simulink model "PX4_Receive"  (R2025b)
settings: Solver=FixedStepAuto  StartTime=0.0  StopTime=60  RelTol=1e-3
undefined symbols (not defined in the file or in its folder): acceleration, actuator, attitude, body_rate, codertarget, command, control, CustomLQR, FlightPlan, from_external, gcbh, HomeNED, HoverThrust, jerk, param1, param2, param3, pitch, pitch_body, position, PX4Params, PX4Tune, q_d, roll, roll_body, source_component, source_system, target_component, target_system, TestAmplitude, TestAxis, thrust_body, timestamp, timestamp_sample, TUNING_ON, TuningMaxClimbRate, TuningMinAltitude, TuningStage, TuningTestStart, velocity, yaw, yaw_body, yaw_sp_move_rate, yawspeed
libraries: px4Utilslib x53, px4uORBlib x52, simulink x13
(part 1 of 2)
settings Model: SimulationMode=external  ExtModeTrigDuration=10  Creator=MarkusKennoHansen  LastModifiedBy=marku
settings SolverCC: PositivePriorityOrder=on  AutoInsertRateTranBlk=on
settings DataIOCC: ReturnWorkspaceOutputs=off
settings OptimizationCC: BlockReduction=off  BooleanDataType=off  EnhancedBackFolding=on  PassReuseOutputArgsAs=Individual arguments  ZeroExternalMemoryAtStartup=off  ZeroInternalMemoryAtStartup=off  MaxStackSize=64  OptimizeBlockOrder=speed  DifferentSizesBufferReuse=on  OptimizationCustomize=off  EfficientTunableParamExpr=on
settings DebuggingCC: SaveWithParameterizedLinksMsg=none  UnderspecifiedInitializationDetection=Classic  MergeDetectMultiDrivingBlocksExec=none  SignalResolutionControl=TryResolveAllWithWarning  IntegerOverflowMsg=none  ParameterPrecisionLossMsg=none  ParameterTunabilityLossMsg=error  IntegerSaturationMsg=none
settings HardwareCC: ProdBitPerPointer=32.0  ProdBitPerSizeT=32.0  ProdBitPerPtrDiffT=32.0  ProdLargestAtomicInteger=Long  ProdLargestAtomicFloat=Double  ProdWordSize=32.0  ProdLongLongMode=on  ProdHWDeviceType=ARM Compatible->ARM Cortex
settings ModelReferenceCC: EnableParallelModelReferenceBuilds=on  PropagateSignalLabelsOutOfModel=off
settings SFSimCC: MATLABDynamicMemAlloc=off  SimTargetLang=C++  SimDLTargetLibrary=mkl-dnn
settings RTWCC: SystemTargetFile=ert.tlc  HardwareBoard=PX4 Host Target  TemplateMakefile=ert_default_tmf  Toolchain=GNU Tools for PX4 Autopilots  PortableWordSizes=on  TargetLang=C++  Description=Embedded Coder
settings CodeAppCC: ForceParamTrailComments=on  IgnoreCustomStorageClasses=off  OperatorAnnotations=on  SimulinkDataObjDesc=on  SFDataObjDesc=on  InsertBlockDesc=on
settings ERTTargetCC: ExtMode=on  ExtModeTransport=2.0  ExtModeStaticAlloc=on  ExtModeMexFile=ext_xcp  ExtModeIntrfLevel=Level2 - Open  InlinedParameterPlacement=Hierarchical

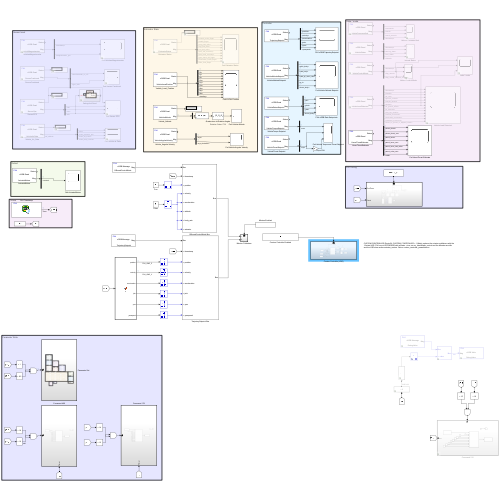
[thumbnail: Simulink's stored preview of the top-level diagram]
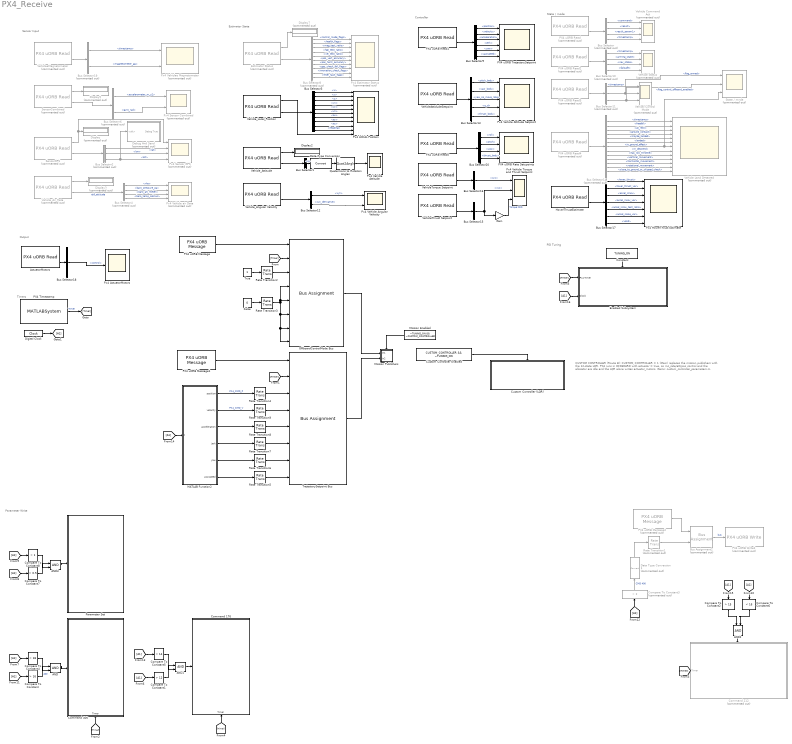
== system PX4_Receive ==
  note: PID Tuning
  note: Timers
  note: Parameter Write
  note: Output
  note: State / mode
  note: Controller
  note: Estimator State
  note: Sensor Input
  note: CUSTOM CONTROLLER (Route B): CUSTOM_CONTROLLER = 1 (Main) replaces the mission publishers with the
      | 12-state LQR. PX4 runs in OFFBOARD with actuator = true, so mc_rate/att/pos_control and the allocator are idle
      | and the LQR alone writes actuator_motors. Gains: custom_controller_parameters.m.
  AND{,1..3} (4 alike) : Logic  IconShape=distinctive  AllPortsSameDT=off  OutDataTypeStr=boolean
  ActuatorMotors : px4uORBlib/PX4 uORB Read  uORBTopic=ActuatorMotors  selectInstance=ActuatorMotors  SampleTime=-1  BlockingMode=off  BlockTimeout=1e-3
  Bus Assignment2 : BusAssignment  Commented=on  AssignedSignals=value
  Bus Selector : BusSelector  Commented=on  OutputSignals=command,result,result_param1,timestamp
  Bus Selector1 : BusSelector  OutputSignals=q
  Bus Selector10 : BusSelector  Commented=on  OutputSignals=timestamp,arming_state,nav_state,failsafe
  Bus Selector11 : BusSelector  Commented=on  OutputSignals=timestamp,flag_armed,flag_control_offboard_enabled
  Bus Selector12 : BusSelector  OutputSignals=xyz,xyz_derivative
  Bus Selector13 : BusSelector  OutputSignals=pitch_body,yaw_body,yaw_sp_move_rate,q_d,thrust_body
  Bus Selector14 : BusSelector  Commented=on  OutputSignals=timestamp,freefall,at_rest,ground_contact,maybe_landed,landed,in_ground_effect,in_descend,has_low_throttle,vertical_movement,horizontal_movement,rotational_movement,close_to_ground_or_skipped_check
  Bus Selector15 : BusSelector  OutputSignals=xyz
  Bus Selector16 : BusSelector  OutputSignals=xyz
  Bus Selector17 : BusSelector  OutputSignals=hover_thrust,hover_thrust_var,accel_innov,accel_innov_var,accel_innov_test_ratio,accel_noise_var,valid
  Bus Selector18 : BusSelector  OutputSignals=control
  Bus Selector19 : BusSelector  Commented=on  OutputSignals=timestamp,magnetometer_ga
  Bus Selector2 : BusSelector  Commented=on  OutputSignals=lat,lon,alt
  Bus Selector20 : BusSelector  OutputSignals=roll,pitch,yaw,thrust_body
  Bus Selector3 : BusSelector  OutputSignals=x,y,z,vx,vy,vz,ax,ay,az,heading
  Bus Selector4 : BusSelector  Commented=on  OutputSignals=rho,baro_pressure_pa,baro_alt_meter,baro_temp_celcius
  Bus Selector6 : BusSelector  Commented=on  OutputSignals=accelerometer_m_s2,gyro_rad
  Bus Selector8 : BusSelector  Commented=on  OutputSignals=control_mode_flags,health_flags,mag_test_ratio,hgt_test_ratio,vel_test_ratio,pos_vert_accuracy,pos_horiz_accuracy,gps_check_fail_flags,innovation_check_flags,filter_fault_flags
  Bus Selector9 : BusSelector  OutputSignals=position,velocity,acceleration,jerk,yaw,yawspeed
  Command 176 : Subsystem
  Command 212 : Subsystem  Commented=on
  Command 400 : Subsystem
  Compare To Constant : simulink/Logic and Bit Operations/Compare To Constant  relop=>  const=16  OutDataTypeStr=boolean
  Compare To Constant1 : simulink/Logic and Bit Operations/Compare To Constant  relop=>  const=12  OutDataTypeStr=boolean
  Compare To Constant2 : simulink/Logic and Bit Operations/Compare To Constant  relop=>  const=15  OutDataTypeStr=boolean
  Compare To Constant3 : simulink/Logic and Bit Operations/Compare To Constant  Commented=on  relop=>  const=2  OutDataTypeStr=boolean
  Compare To Constant4 : simulink/Logic and Bit Operations/Compare To Constant  relop=<  const=18  OutDataTypeStr=boolean
  Compare To Constant5 : simulink/Logic and Bit Operations/Compare To Constant  relop=<  const=14  OutDataTypeStr=boolean
  Compare To Constant6 : simulink/Logic and Bit Operations/Compare To Constant  relop=<  const=16  OutDataTypeStr=boolean
  Compare To Constant7 : simulink/Logic and Bit Operations/Compare To Constant  relop=>  const=0.5  OutDataTypeStr=boolean
  Compare To Constant8 : simulink/Logic and Bit Operations/Compare To Constant  relop=<  const=1  OutDataTypeStr=boolean
  Constant : Constant  Value=TUNING_ON
  Custom Controller (LQR) : Subsystem
  Custom Controller Enabled : Constant  Value=CUSTOM_CONTROLLER && ~TUNING_ON  OutDataTypeStr=boolean
  Data Type Conversion : DataTypeConversion  SaturateOnIntegerOverflow=off  RndMeth=Floor
  Data Type Conversion1 : DataTypeConversion  Commented=on  SaturateOnIntegerOverflow=off  RndMeth=Floor
  Debug And Send : Subsystem  Commented=on
  Digital Clock : DigitalClock  SampleTime=0.01
  Display{,3,5,7} (4 alike) : Display  Commented=on
  Display2 : Display
  Enabled Subsystem : Subsystem  TreatAsAtomicUnit=on
  Estimator Status : px4uORBlib/PX4 uORB Read  Commented=on  uORBTopic=EstimatorStatus  selectInstance=EstimatorStatus  SampleTime=-1  BlockingMode=off  BlockTimeout=1e-3
  False : Constant  Value=0  OutDataTypeStr=Inherit: Inherit via back propagation
  Gain : Gain  Gain=[1 -1 -1]
  HoverThrustEstimate : px4uORBlib/PX4 uORB Read  uORBTopic=HoverThrustEstimate  selectInstance=HoverThrustEstimate  SampleTime=-1  BlockingMode=off  BlockTimeout=1e-3
  MATLAB Function2 : MATLAB Function  TreatAsAtomicUnit=on
  Mission Enabled : Constant  Value=~TUNING_ON && ~CUSTOM_CONTROLLER  OutDataTypeStr=boolean
  Mission Publishers : Subsystem
  OffboardControlMode Bus : BusAssignment  AssignedSignals=timestamp,position,velocity,acceleration,attitude,body_rate,actuator
  PX4 Timestamp : MATLABSystem  InitFcn=codertarget.pixhawk.internal.registration.registerBlockInResourceMgr(gcbh,'PX4_Timestamp');  System=px4.internal.block.getPX4AbsoluteTime  SampleTime=0.01
  PX4 uORB Message : px4uORBlib/PX4 uORB Message  uORBTopic=OffboardControlMode  SampleTime=-1  selectInstance=OffboardControlMode
  PX4 uORB Message1 : px4uORBlib/PX4 uORB Message  uORBTopic=TrajectorySetpoint  SampleTime=-1  selectInstance=TrajectorySetpoint
  PX4 uORB Message2 : px4uORBlib/PX4 uORB Message  Commented=on  uORBTopic=DebugValue  SampleTime=-1  selectInstance=DebugValue
  PX4 uORB Rate Setupoints : Scope  NumInputPorts=4
      settings: ActiveDisplayYMinimum=-4.7996553778648376  ActiveDisplayYMaximum=4.7996553778648376  DataLoggingVariableName=ScopeData22
  PX4 uORB Read : px4uORBlib/PX4 uORB Read  Commented=on  uORBTopic=VehicleCommandAck  selectInstance=VehicleCommandAck  SampleTime=-1  BlockingMode=off  BlockTimeout=1e-3
  PX4 uORB Read1 : px4uORBlib/PX4 uORB Read  uORBTopic=TrajectorySetpoint  selectInstance=TrajectorySetpoint  SampleTime=-1  BlockingMode=off  BlockTimeout=1e-3
  PX4 uORB Read2 : px4uORBlib/PX4 uORB Read  Commented=on  uORBTopic=VehicleStatus  selectInstance=VehicleStatus  SampleTime=-1  BlockingMode=off  BlockTimeout=1e-3
  PX4 uORB Read3 : px4uORBlib/PX4 uORB Read  Commented=on  uORBTopic=VehicleControlMode  selectInstance=VehicleControlMode  SampleTime=-1  BlockingMode=off  BlockTimeout=1e-3
  PX4 uORB Read4 : px4uORBlib/PX4 uORB Read  Commented=on  uORBTopic=VehicleLandDetected  selectInstance=VehicleLandDetected  SampleTime=-1  BlockingMode=off  BlockTimeout=1e-3
  PX4 uORB Read5 : px4uORBlib/PX4 uORB Read  uORBTopic=VehicleRatesSetpoint  selectInstance=VehicleRatesSetpoint  SampleTime=-1  BlockingMode=off  BlockTimeout=1e-3
  PX4 uORB TrajectorySetpoint : Scope  NumInputPorts=6
      settings: ActiveDisplayYMinimum=-0.034024091670289636  ActiveDisplayYMaximum=0.16679841303266585  DataLoggingVariableName=ScopeData13
  PX4 uORB Write2 : px4uORBlib/PX4 uORB Write  Commented=on  uORBTopic=DebugValue  selectInstance=DebugValue  MessageQueueLen=1
  Parameter Set : Subsystem
  Px4 ActuatorMotors : Scope
      settings: ActiveDisplayYMinimum=-0.12499999999999997  ActiveDisplayYMaximum=1.125  DataLoggingVariableName=ScopeData20
  "Px4 Estimator Status " : Scope  Commented=on  NumInputPorts=10
      settings: ActiveDisplayString=3  ActiveDisplayYMinimum=-0.00022157638159114862  ActiveDisplayYMaximum=0.0019941874343203381  DataLoggingVariableName=ScopeData7
  Px4 HoverThrust Estimate : Scope  NumInputPorts=7
      settings: ActiveDisplayYMinimum=-1  ActiveDisplayYMaximum=1  DataLoggingVariableName=ScopeData19
  Px4 LOCAL Position : Scope  NumInputPorts=11
      settings: ActiveDisplayYMinimum=-0.0066038075601682067  ActiveDisplayYMaximum=0.015251552104018629  DataLoggingVariableName=ScopeData3
  Px4 Sensor Combined : Scope  Commented=on  NumInputPorts=2
      settings: ActiveDisplayYMinimum=-34.435865640640259  ActiveDisplayYMaximum=33.0942919254303  DataLoggingVariableName=ScopeData6
  Px4 Sensor GPS : Scope  Commented=on  NumInputPorts=4
      settings: ActiveDisplayString=3  ActiveDisplayYMinimum=1.25208830125E+8  ActiveDisplayYMaximum=1.25210948875E+8
  Px4 Vehiclae Magnetometer : Scope  Commented=on  NumInputPorts=2
      settings: ActiveDisplayYMinimum=-0.399243738502264  ActiveDisplayYMaximum=0.3986239992082119  DataLoggingVariableName=ScopeData21
  Px4 Vehicle Angular Velocity : Scope  NumInputPorts=2
      settings: ActiveDisplayYMinimum=-617.98886871337891  ActiveDisplayYMaximum=742.34903717041016  DataLoggingVariableName=ScopeData15
  Px4 Vehicle Attitude : Scope
      settings: ActiveDisplayYMinimum=-3.9110912623215079  ActiveDisplayYMaximum=3.91992136617894  DataLoggingVariableName=ScopeData2
  Px4 Vehicle Attitude Setpoint : Scope  NumInputPorts=5
      settings: ActiveDisplayYMinimum=1.739683210849762  ActiveDisplayYMaximum=1.742851197719574  DataLoggingVariableName=ScopeData16
  Px4 Vehicle Torque and Thrust Setpoint : Scope  NumInputPorts=3
      settings: ActiveDisplayYMinimum=-0.20918363705277443  ActiveDisplayYMaximum=0.023242626339197155  DataLoggingVariableName=ScopeData18
  Px4 Vehicle air Data : Scope  Commented=on  NumInputPorts=4
      settings: ActiveDisplayString=3  ActiveDisplayYMinimum=0.95836924761533737  ActiveDisplayYMaximum=0.99945063143968582  DataLoggingVariableName=ScopeData4
  Quaternions to Rotation Angles : Quat2Angle
      settings: AttributesFormatString=Rotation Order: %<rotationOrder>
  Rate Transition1 : RateTransition  Commented=on  OutPortSampleTime=1/500
  Rate Transition{2..9} (8 alike) : RateTransition  Deterministic=off  OutPortSampleTime=0.01
  SensorCombined : px4uORBlib/PX4 uORB Read  Commented=on  uORBTopic=SensorCombined  selectInstance=SensorCombined  SampleTime=-1  BlockingMode=off  BlockTimeout=1e-3
  SensorGPS : px4uORBlib/PX4 uORB Read  Commented=on  uORBTopic=SensorGps  selectInstance=sensor_gps  SampleTime=-1  BlockingMode=off  BlockTimeout=1e-3
  State / mode : Scope  Commented=on  NumInputPorts=3
      settings: DataLoggingVariableName=ScopeData23
  TrajectorySetpoint Bus : BusAssignment  AssignedSignals=timestamp,position,velocity,acceleration,jerk,yaw,yawspeed
  True : Constant  OutDataTypeStr=Inherit: Inherit via back propagation
  Vehical Control Mode : Scope  Commented=on  NumInputPorts=3
      settings: ActiveDisplayYMinimum=3.7235000000000009E+6  ActiveDisplayYMaximum=4.56485E+7  DataLoggingVariableName=ScopeData14
  Vehical Status : Scope  Commented=on  NumInputPorts=4
      settings: ActiveDisplayYMinimum=833500.00000000093  ActiveDisplayYMaximum=3.56185E+7  DataLoggingVariableName=ScopeData8
  VehiclaeMagnetometer : px4uORBlib/PX4 uORB Read  Commented=on  uORBTopic=VehicleMagnetometer  selectInstance=VehicleMagnetometer  SampleTime=-1  BlockingMode=off  BlockTimeout=1e-3
  Vehicle Command Ack : Scope  Commented=on  NumInputPorts=4
      settings: ActiveDisplayYMinimum=-49.999999999999986  ActiveDisplayYMaximum=450  DataLoggingVariableName=ScopeData12
  Vehicle Land Detected : Scope  Commented=on  NumInputPorts=13
      settings: ActiveDisplayYMinimum=3.0415000000000009E+6  ActiveDisplayYMaximum=4.55065E+7  DataLoggingVariableName=ScopeData17
  VehicleAttidudeSetpoint : px4uORBlib/PX4 uORB Read  uORBTopic=VehicleAttitudeSetpoint  selectInstance=vehicle_attitude_setpoint  SampleTime=-1  BlockingMode=off  BlockTimeout=1e-3
  VehicleThrust Setpoint : px4uORBlib/PX4 uORB Read  uORBTopic=VehicleThrustSetpoint  selectInstance=vehicle_thrust_setpoint  SampleTime=-1  BlockingMode=off  BlockTimeout=1e-3
  VehicleTorque Setpoint : px4uORBlib/PX4 uORB Read  uORBTopic=VehicleTorqueSetpoint  selectInstance=vehicle_torque_setpoint  SampleTime=-1  BlockingMode=off  BlockTimeout=1e-3
  Vehicle_Air_Data : px4uORBlib/PX4 uORB Read  Commented=on  uORBTopic=VehicleAirData  selectInstance=VehicleAirData  SampleTime=-1  BlockingMode=off  BlockTimeout=1e-3
  Vehicle_Angular Velocity : px4uORBlib/PX4 uORB Read  uORBTopic=VehicleAngularVelocity  selectInstance=vehicle_angular_velocity  SampleTime=-1  BlockingMode=off  BlockTimeout=1e-3
  Vehicle_Attitude : px4uORBlib/PX4 uORB Read  uORBTopic=VehicleAttitude  selectInstance=vehicle_attitude  SampleTime=-1  BlockingMode=off  BlockTimeout=1e-3
  Vehicle_Local_Position : px4uORBlib/PX4 uORB Read  uORBTopic=VehicleLocalPosition  selectInstance=vehicle_local_position  SampleTime=-1  BlockingMode=off  BlockTimeout=1e-3
  wires:
  Bus Selector2/2 -> Px4 Sensor GPS/3  "<lon>"
  Bus Selector2/3 -> Px4 Sensor GPS/4, Debug And Send/1(<alt>)  "<alt>"
  Bus Selector2/1 -> Px4 Sensor GPS/2  "<lat>"
  SensorGPS/1 -> Display/1, Px4 Sensor GPS/1
  SensorGPS/2 -> Bus Selector2/1
  Vehicle_Attitude/2 -> Bus Selector1/1
  Vehicle_Local_Position/2 -> Bus Selector3/1
  Bus Selector1/1 -> Data Type Conversion/1  "<q>"
  Quaternions to Rotation Angles/1 -> Px4 Vehicle Attitude/1
  Data Type Conversion/1 -> Quaternions to Rotation Angles/1
  Vehicle_Attitude/1 -> Display2/1
  Rate Transition2/1 -> OffboardControlMode Bus/3
  Rate Transition9/1 -> TrajectorySetpoint Bus/4
  Rate Transition7/1 -> TrajectorySetpoint Bus/6
  Rate Transition4/1 -> TrajectorySetpoint Bus/3
  PX4 uORB Message1/1 -> TrajectorySetpoint Bus/1
  False/1 -> Rate Transition3/1
  PX4 uORB Message/1 -> OffboardControlMode Bus/1
  MATLAB Function2/4(jerk) -> Rate Transition7/1
  True/1 -> Rate Transition2/1
  Rate Transition5/1 -> TrajectorySetpoint Bus/8
  Rate Transition3/1 -> OffboardControlMode Bus/7, OffboardControlMode Bus/8, OffboardControlMode Bus/6, OffboardControlMode Bus/4, OffboardControlMode Bus/5
  Rate Transition6/1 -> TrajectorySetpoint Bus/7
  Rate Transition8/1 -> TrajectorySetpoint Bus/5
  PX4 uORB Read/2 -> Bus Selector/1
  Bus Selector/1 -> Vehicle Command Ack/1  "<command>"
  Bus Selector/2 -> Vehicle Command Ack/2  "<result>"
  Bus Selector/3 -> Vehicle Command Ack/3  "<result_param1>"
  Bus Selector/4 -> Vehicle Command Ack/4  "<timestamp>"
  Bus Assignment2/1 -> PX4 uORB Write2/1  "bus"
  PX4 uORB Message2/1 -> Bus Assignment2/1
  Rate Transition1/1 -> Bus Assignment2/2
  Data Type Conversion1/1 -> Rate Transition1/1
  PX4 uORB Read1/2 -> Bus Selector9/1
  Bus Selector9/1 -> PX4 uORB TrajectorySetpoint/1  "<position>"
  Bus Selector9/2 -> PX4 uORB TrajectorySetpoint/2  "<velocity>"
  Bus Selector9/3 -> PX4 uORB TrajectorySetpoint/3  "<acceleration>"
  Bus Selector9/4 -> PX4 uORB TrajectorySetpoint/4  "<jerk>"
  Bus Selector9/5 -> PX4 uORB TrajectorySetpoint/5  "<yaw>"
  Bus Selector9/6 -> PX4 uORB TrajectorySetpoint/6  "<yawspeed>"
  Compare To Constant3/1 -> Data Type Conversion1/1  "CMD 400"
  AND/1 -> Command 400/Trigger
  Compare To Constant/1 -> AND/1  "400"
  Compare To Constant4/1 -> AND/2
  AND1/1 -> Command 176/Trigger
  Compare To Constant1/1 -> AND1/1
  Compare To Constant5/1 -> AND1/2
  Compare To Constant2/1 -> AND2/1
  AND2/1 -> Command 212/Trigger
  Compare To Constant6/1 -> AND2/2
  Compare To Constant7/1 -> AND3/1
  Compare To Constant8/1 -> AND3/2
  AND3/1 -> Parameter Set/Trigger
  PX4 uORB Read2/2 -> Bus Selector10/1
  Bus Selector10/1 -> Vehical Status/1  "<timestamp>"
  Bus Selector10/3 -> Vehical Status/3  "<nav_state>"
  Bus Selector10/4 -> Vehical Status/4  "<failsafe>"
  PX4 uORB Read3/2 -> Bus Selector11/1
  Bus Selector10/2 -> Vehical Status/2  "<arming_state>"
  Bus Selector11/1 -> Vehical Control Mode/1  "<timestamp>"
  Bus Selector11/2 -> State / mode/1, Vehical Control Mode/2  "<flag_armed>"
  Bus Selector11/3 -> State / mode/2, Vehical Control Mode/3  "<flag_control_offboard_enabled>"
  Vehicle_Angular Velocity/2 -> Bus Selector12/1
  Bus Selector12/1 -> Px4 Vehicle Angular Velocity/1  "<xyz>"
  Bus Selector12/2 -> Px4 Vehicle Angular Velocity/2  "<xyz_derivative>"
  VehicleAttidudeSetpoint/2 -> Bus Selector13/1
  Bus Selector13/1 -> Px4 Vehicle Attitude Setpoint/1  "<pitch_body>"
  Bus Selector13/2 -> Px4 Vehicle Attitude Setpoint/2  "<yaw_body>"
  Bus Selector13/3 -> Px4 Vehicle Attitude Setpoint/3  "<yaw_sp_move_rate>"
  Bus Selector13/4 -> Px4 Vehicle Attitude Setpoint/4  "<q_d>"
  Bus Selector13/5 -> Px4 Vehicle Attitude Setpoint/5  "<thrust_body>"
  PX4 uORB Read4/2 -> Bus Selector14/1
  Bus Selector14/1 -> Vehicle Land Detected/1  "<timestamp>"
  Bus Selector14/2 -> Vehicle Land Detected/2  "<freefall>"
  Bus Selector14/3 -> Vehicle Land Detected/3  "<at_rest>"
  Bus Selector14/4 -> Vehicle Land Detected/4  "<ground_contact>"
  Bus Selector14/5 -> Vehicle Land Detected/5  "<maybe_landed>"
  Bus Selector14/6 -> Vehicle Land Detected/6  "<landed>"
  Bus Selector14/7 -> State / mode/3, Vehicle Land Detected/7  "<in_ground_effect>"
  Bus Selector14/8 -> Vehicle Land Detected/8  "<in_descend>"
  Bus Selector14/9 -> Vehicle Land Detected/9  "<has_low_throttle>"
  Bus Selector14/10 -> Vehicle Land Detected/10  "<vertical_movement>"
  Bus Selector14/11 -> Vehicle Land Detected/11  "<horizontal_movement>"
  Bus Selector14/12 -> Vehicle Land Detected/12  "<rotational_movement>"
  Bus Selector14/13 -> Vehicle Land Detected/13  "<close_to_ground_or_skipped_check>"
  VehicleThrust Setpoint/2 -> Bus Selector15/1
  VehicleTorque Setpoint/2 -> Bus Selector16/1
  HoverThrustEstimate/2 -> Bus Selector17/1
  Bus Selector16/1 -> Px4 Vehicle Torque and Thrust Setpoint/1  "<xyz>"
  Bus Selector15/1 -> Gain/1, Px4 Vehicle Torque and Thrust Setpoint/2  "<xyz>"
  Bus Selector17/1 -> Px4 HoverThrust Estimate/1  "<hover_thrust>"
  Bus Selector17/2 -> Px4 HoverThrust Estimate/2  "<hover_thrust_var>"
  Bus Selector17/3 -> Px4 HoverThrust Estimate/3  "<accel_innov>"
  Bus Selector17/4 -> Px4 HoverThrust Estimate/4  "<accel_innov_var>"
  Bus Selector17/5 -> Px4 HoverThrust Estimate/5  "<accel_innov_test_ratio>"
  Bus Selector17/6 -> Px4 HoverThrust Estimate/6  "<accel_noise_var>"
  Bus Selector17/7 -> Px4 HoverThrust Estimate/7  "<valid>"
  Bus Selector6/1 -> Px4 Sensor Combined/1  "<accelerometer_m_s2>"
  Bus Selector6/2 -> Px4 Sensor Combined/2  "<gyro_rad>"
  SensorCombined/1 -> Display5/1
  SensorCombined/2 -> Bus Selector6/1
  ActuatorMotors/2 -> Bus Selector18/1
  VehiclaeMagnetometer/2 -> Bus Selector19/1
  Bus Selector19/1 -> Px4 Vehiclae Magnetometer/1  "<timestamp>"
  Bus Selector19/2 -> Px4 Vehiclae Magnetometer/2  "<magnetometer_ga>"
  Bus Selector4/2 -> Px4 Vehicle air Data/2  "<baro_pressure_pa>"
  Vehicle_Air_Data/2 -> Bus Selector4/1  "ekf_attitude"
  Bus Selector4/3 -> Px4 Vehicle air Data/3  "<baro_alt_meter>"
  Vehicle_Air_Data/1 -> Display3/1
  Bus Selector4/4 -> Px4 Vehicle air Data/4  "<baro_temp_celcius>"
  Bus Selector4/1 -> Px4 Vehicle air Data/1  "<rho>"
  Bus Selector8/10 -> "Px4 Estimator Status "/10  "<filter_fault_flags>"
  Bus Selector8/8 -> "Px4 Estimator Status "/8  "<gps_check_fail_flags>"
  Bus Selector8/9 -> "Px4 Estimator Status "/9  "<innovation_check_flags>"
  Estimator Status/2 -> Bus Selector8/1
  Estimator Status/1 -> Display7/1
  Bus Selector8/1 -> "Px4 Estimator Status "/1  "<control_mode_flags>"
  Bus Selector8/5 -> "Px4 Estimator Status "/5  "<vel_test_ratio>"
  Bus Selector8/3 -> "Px4 Estimator Status "/3  "<mag_test_ratio>"
  Bus Selector8/7 -> "Px4 Estimator Status "/7  "<pos_horiz_accuracy>"
  Bus Selector8/6 -> "Px4 Estimator Status "/6  "<pos_vert_accuracy>"
  Bus Selector8/4 -> "Px4 Estimator Status "/4  "<hgt_test_ratio>"
  Bus Selector8/2 -> "Px4 Estimator Status "/2  "<health_flags>"
  PX4 uORB Read5/2 -> Bus Selector20/1
  Bus Selector20/1 -> PX4 uORB Rate Setupoints/1  "<roll>"
  Bus Selector20/2 -> PX4 uORB Rate Setupoints/2  "<pitch>"
  Bus Selector20/3 -> PX4 uORB Rate Setupoints/3  "<yaw>"
  Bus Selector20/4 -> PX4 uORB Rate Setupoints/4  "<thrust_body>"
  Bus Selector18/1 -> Px4 ActuatorMotors/1  "<control>"
  Gain/1 -> Px4 Vehicle Torque and Thrust Setpoint/3  "Torque FRD"
  MATLAB Function2/1(position) -> Rate Transition4/1  "PX4_CMD_P"
  Bus Selector3/1 -> Px4 LOCAL Position/1  "<x>"
  Bus Selector3/2 -> Px4 LOCAL Position/2  "<y>"
  Bus Selector3/3 -> Px4 LOCAL Position/3  "<z>"
  Bus Selector3/4 -> Px4 LOCAL Position/4  "<vx>"
  Bus Selector3/5 -> Px4 LOCAL Position/5  "<vy>"
  Bus Selector3/6 -> Px4 LOCAL Position/6  "<vz>"
  Bus Selector3/7 -> Px4 LOCAL Position/7  "<ax>"
  Bus Selector3/8 -> Px4 LOCAL Position/8  "<ay>"
  Bus Selector3/9 -> Px4 LOCAL Position/9  "<az>"
  Bus Selector3/10 -> Px4 LOCAL Position/10  "<heading>"
  Vehicle_Local_Position/1 -> Px4 LOCAL Position/11
  MATLAB Function2/2(velocity) -> Rate Transition9/1  "PX4_CMD_V"
  MATLAB Function2/3(acceleration) -> Rate Transition8/1
  MATLAB Function2/5(yaw) -> Rate Transition6/1
  MATLAB Function2/6(yawspeed) -> Rate Transition5/1
  Constant/1 -> Enabled Subsystem/Enable
  PX4 Timestamp/1 -> [Timer]  "Timer"
  [Timer] -> OffboardControlMode Bus/2
  [Timer] -> TrajectorySetpoint Bus/2
  [Timer] -> Command 400/1(Timer)
  [Timer] -> Command 212/1(Timer)
  [Timer] -> Command 176/1(Timer)
  [Timer] -> Enabled Subsystem/1(Px4 Timer)
  Digital Clock/1 -> [A1]
  [A1] -> Compare To Constant1/1
  [A1] -> Compare To Constant4/1
  [A1] -> Compare To Constant7/1
  [A1] -> Compare To Constant8/1
  [A1] -> Compare To Constant6/1
  [A1] -> Compare To Constant/1
  [A1] -> Compare To Constant3/1
  [A1] -> Compare To Constant5/1
  [A1] -> MATLAB Function2/1(t)
  [A1] -> Compare To Constant2/1
  [A1] -> Enabled Subsystem/2(Clock)
  OffboardControlMode Bus/1 -> Mission Publishers/1(In1)
  TrajectorySetpoint Bus/1 -> Mission Publishers/2(In2)
  Mission Enabled/1 -> Mission Publishers/Enable
  Custom Controller Enabled/1 -> Custom Controller (LQR)/Enable

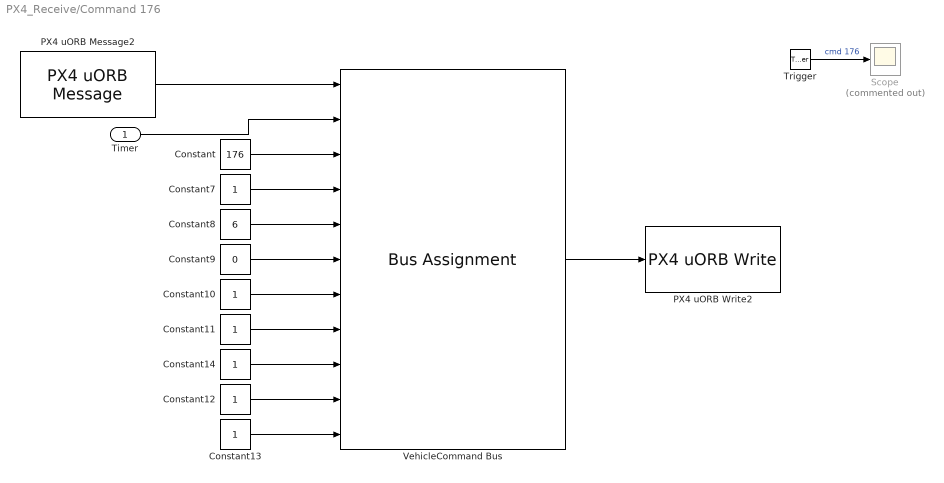
== system PX4_Receive/Command 176 ==
  Timer : Inport
  Trigger : TriggerPort  VariantControl=(inherit)  ShowOutputPort=on  PortDimensions=1
  Constant : Constant  Value=176  OutDataTypeStr=Inherit: Inherit via back propagation  SampleTime=-1
  Constant{7,10..14} (6 alike) : Constant  OutDataTypeStr=Inherit: Inherit via back propagation  SampleTime=-1
  Constant8 : Constant  Value=6  OutDataTypeStr=Inherit: Inherit via back propagation  SampleTime=-1
  Constant9 : Constant  Value=0  OutDataTypeStr=Inherit: Inherit via back propagation  SampleTime=-1
  PX4 uORB Message2 : px4uORBlib/PX4 uORB Message  uORBTopic=VehicleCommand  SampleTime=-1  selectInstance=vehicle_command
  PX4 uORB Write2 : px4uORBlib/PX4 uORB Write  uORBTopic=VehicleCommand  selectInstance=vehicle_command  MessageQueueLen=1
  Scope : Scope  Commented=on
      settings: ActiveDisplayYMinimum=-0.12499999999999997  ActiveDisplayYMaximum=1.125  DataLoggingVariableName=ScopeData10
  VehicleCommand Bus : BusAssignment  AssignedSignals=timestamp,command,param1,param2,param3,target_system,target_component,source_system,source_component,from_external
  wires:
  Constant7/1 -> VehicleCommand Bus/4
  Constant12/1 -> VehicleCommand Bus/10
  Constant11/1 -> VehicleCommand Bus/8
  Constant10/1 -> VehicleCommand Bus/7
  VehicleCommand Bus/1 -> PX4 uORB Write2/1
  Constant14/1 -> VehicleCommand Bus/9
  Constant13/1 -> VehicleCommand Bus/11
  Constant8/1 -> VehicleCommand Bus/5
  PX4 uORB Message2/1 -> VehicleCommand Bus/1
  Constant9/1 -> VehicleCommand Bus/6
  Constant/1 -> VehicleCommand Bus/3
  Trigger/1 -> Scope/1  "cmd 176"
  Timer/1 -> VehicleCommand Bus/2

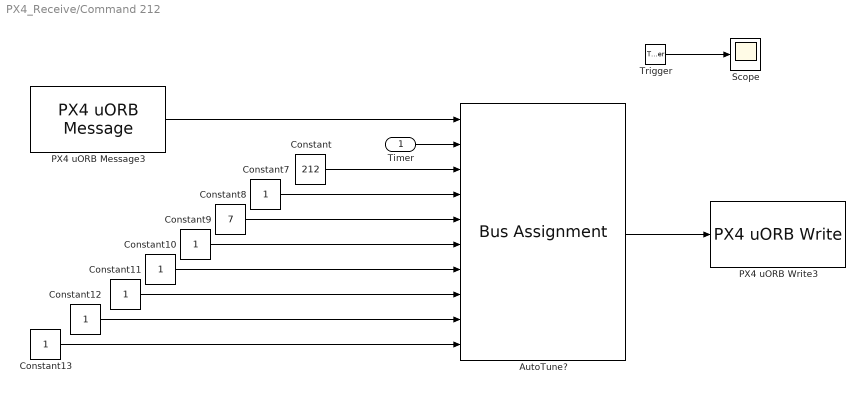
== system PX4_Receive/Command 212 ==
  Timer : Inport
  Trigger : TriggerPort  VariantControl=(inherit)  ShowOutputPort=on  PortDimensions=1
  AutoTune? : BusAssignment  AssignedSignals=timestamp,command,param1,param2,target_system,target_component,source_system,source_component,from_external
  Constant : Constant  Value=212  OutDataTypeStr=Inherit: Inherit via back propagation
  Constant{7,9..13} (6 alike) : Constant  OutDataTypeStr=Inherit: Inherit via back propagation
  Constant8 : Constant  Value=7  OutDataTypeStr=Inherit: Inherit via back propagation
  PX4 uORB Message3 : px4uORBlib/PX4 uORB Message  uORBTopic=VehicleCommand  SampleTime=-1  selectInstance=vehicle_command
  PX4 uORB Write3 : px4uORBlib/PX4 uORB Write  uORBTopic=VehicleCommand  selectInstance=vehicle_command  MessageQueueLen=1
  Scope : Scope
      settings: ActiveDisplayYMinimum=-0.12499999999999997  ActiveDisplayYMaximum=1.125  DataLoggingVariableName=ScopeData11
  wires:
  Trigger/1 -> Scope/1
  Constant12/1 -> AutoTune?/9
  Constant7/1 -> AutoTune?/4
  Constant10/1 -> AutoTune?/7
  Constant8/1 -> AutoTune?/5
  PX4 uORB Message3/1 -> AutoTune?/1
  Constant/1 -> AutoTune?/3
  Constant11/1 -> AutoTune?/8
  Constant9/1 -> AutoTune?/6
  AutoTune?/1 -> PX4 uORB Write3/1
  Constant13/1 -> AutoTune?/10
  Timer/1 -> AutoTune?/2

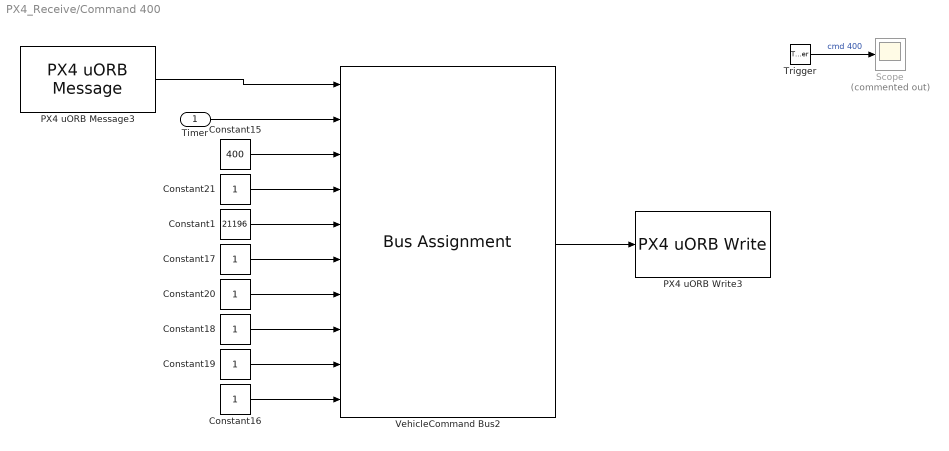
== system PX4_Receive/Command 400 ==
  Timer : Inport
  Trigger : TriggerPort  VariantControl=(inherit)  ShowOutputPort=on  PortDimensions=1
  Constant1 : Constant  Value=21196  OutDataTypeStr=Inherit: Inherit via back propagation  SampleTime=-1
  Constant15 : Constant  Value=400  OutDataTypeStr=Inherit: Inherit via back propagation  SampleTime=-1
  Constant{16..21} (6 alike) : Constant  OutDataTypeStr=Inherit: Inherit via back propagation  SampleTime=-1
  PX4 uORB Message3 : px4uORBlib/PX4 uORB Message  uORBTopic=VehicleCommand  SampleTime=-1  selectInstance=vehicle_command
  PX4 uORB Write3 : px4uORBlib/PX4 uORB Write  uORBTopic=VehicleCommand  selectInstance=vehicle_command  MessageQueueLen=1
  Scope : Scope  Commented=on
      settings: ActiveDisplayYMinimum=-0.12499999999999997  ActiveDisplayYMaximum=1.125  DataLoggingVariableName=ScopeData11
  VehicleCommand Bus2 : BusAssignment  AssignedSignals=timestamp,command,param1,param2,target_system,target_component,source_system,source_component,from_external
  wires:
  Constant21/1 -> VehicleCommand Bus2/4
  PX4 uORB Message3/1 -> VehicleCommand Bus2/1
  VehicleCommand Bus2/1 -> PX4 uORB Write3/1
  Constant17/1 -> VehicleCommand Bus2/6
  Constant20/1 -> VehicleCommand Bus2/7
  Constant19/1 -> VehicleCommand Bus2/9
  Constant18/1 -> VehicleCommand Bus2/8
  Constant15/1 -> VehicleCommand Bus2/3
  Constant16/1 -> VehicleCommand Bus2/10
  Trigger/1 -> Scope/1  "cmd 400"
  Timer/1 -> VehicleCommand Bus2/2
  Constant1/1 -> VehicleCommand Bus2/5

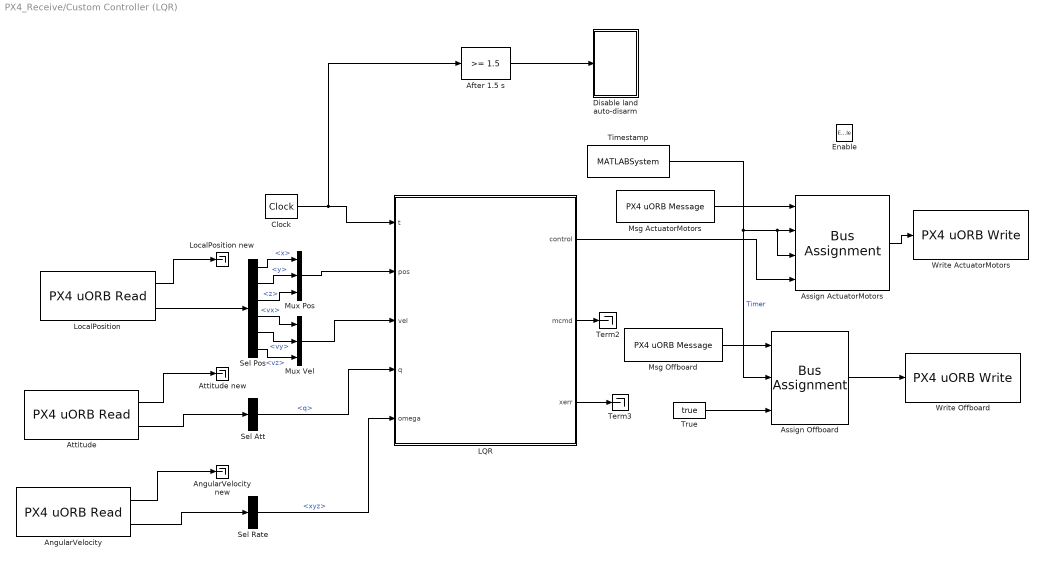
== system PX4_Receive/Custom Controller (LQR) ==
  Enable : EnablePort  StatesWhenEnabling=reset
  After 1.5 s : simulink/Logic and Bit Operations/Compare To Constant  relop=>=  const=1.5  OutDataTypeStr=boolean
  AngularVelocity : px4uORBlib/PX4 uORB Read  uORBTopic=VehicleAngularVelocity  selectInstance=vehicle_angular_velocity  SampleTime=-1  BlockingMode=off  BlockTimeout=1e-3
  AngularVelocity new : Terminator
  Assign ActuatorMotors : BusAssignment  AssignedSignals=timestamp,timestamp_sample,control
  Assign Offboard : BusAssignment  AssignedSignals=timestamp,actuator
  Attitude : px4uORBlib/PX4 uORB Read  uORBTopic=VehicleAttitude  selectInstance=vehicle_attitude  SampleTime=-1  BlockingMode=off  BlockTimeout=1e-3
  Attitude new : Terminator
  Clock : DigitalClock  SampleTime=0.01
  Disable land auto-disarm : Subsystem
  LQR : MATLAB Function  TreatAsAtomicUnit=on
  LocalPosition : px4uORBlib/PX4 uORB Read  uORBTopic=VehicleLocalPosition  selectInstance=vehicle_local_position  SampleTime=-1  BlockingMode=off  BlockTimeout=1e-3
  LocalPosition new : Terminator
  Msg ActuatorMotors : px4uORBlib/PX4 uORB Message  uORBTopic=ActuatorMotors  SampleTime=-1  selectInstance=ActuatorMotors
  Msg Offboard : px4uORBlib/PX4 uORB Message  uORBTopic=OffboardControlMode  SampleTime=-1  selectInstance=OffboardControlMode
  Mux Pos : Mux  Inputs=3
  Mux Vel : Mux  Inputs=3
  Sel Att : BusSelector  OutputSignals=q
  Sel Pos : BusSelector  OutputSignals=x,y,z,vx,vy,vz
  Sel Rate : BusSelector  OutputSignals=xyz
  Term2 : Terminator
  Term3 : Terminator
  Timestamp : MATLABSystem  InitFcn=codertarget.pixhawk.internal.registration.registerBlockInResourceMgr(gcbh,'PX4_Timestamp');  System=px4.internal.block.getPX4AbsoluteTime  SampleTime=0.01
  True : Constant  Value=true  OutDataTypeStr=boolean
  Write ActuatorMotors : px4uORBlib/PX4 uORB Write  uORBTopic=ActuatorMotors  selectInstance=ActuatorMotors  MessageQueueLen=1
  Write Offboard : px4uORBlib/PX4 uORB Write  uORBTopic=OffboardControlMode  selectInstance=OffboardControlMode  MessageQueueLen=1
  wires:
  LocalPosition/1 -> LocalPosition new/1
  Attitude/1 -> Attitude new/1
  AngularVelocity/1 -> AngularVelocity new/1
  LocalPosition/2 -> Sel Pos/1
  Sel Pos/1 -> Mux Pos/1  "<x>"
  Sel Pos/4 -> Mux Vel/1  "<vx>"
  Sel Pos/2 -> Mux Pos/2  "<y>"
  Sel Pos/5 -> Mux Vel/2  "<vy>"
  Sel Pos/3 -> Mux Pos/3  "<z>"
  Sel Pos/6 -> Mux Vel/3  "<vz>"
  Attitude/2 -> Sel Att/1
  AngularVelocity/2 -> Sel Rate/1
  Clock/1 -> LQR/1(t), After 1.5 s/1
  Mux Pos/1 -> LQR/2(pos)
  Mux Vel/1 -> LQR/3(vel)
  Sel Att/1 -> LQR/4(q)  "<q>"
  Sel Rate/1 -> LQR/5(omega)  "<xyz>"
  Msg ActuatorMotors/1 -> Assign ActuatorMotors/1
  Timestamp/1 -> Assign ActuatorMotors/3, Assign ActuatorMotors/2, Assign Offboard/2  "Timer"
  LQR/1(control) -> Assign ActuatorMotors/4
  Assign ActuatorMotors/1 -> Write ActuatorMotors/1
  Msg Offboard/1 -> Assign Offboard/1
  True/1 -> Assign Offboard/3
  Assign Offboard/1 -> Write Offboard/1
  After 1.5 s/1 -> Disable land auto-disarm/Trigger
  LQR/2(mcmd) -> Term2/1
  LQR/3(xerr) -> Term3/1

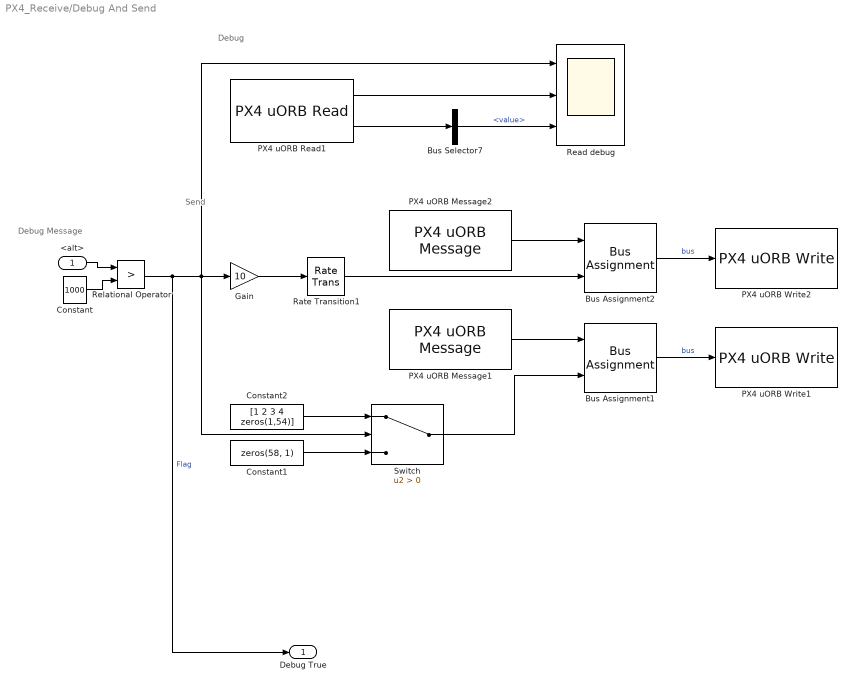
== system PX4_Receive/Debug And Send ==
  note: Send
  note: Debug Message
  note: Debug
  <alt> : Inport
  Bus Assignment1 : BusAssignment  AssignedSignals=data
  Bus Assignment2 : BusAssignment  AssignedSignals=value
  Bus Selector7 : BusSelector  OutputSignals=value
  Constant : Constant  Value=1000  SampleTime=-1
  Constant1 : Constant  Value=zeros(58, 1)  OutDataTypeStr=Inherit: Inherit via back propagation
  Constant2 : Constant  Value=[1 2 3 4 zeros(1,54)]  OutDataTypeStr=Inherit: Inherit via back propagation
  Gain : Gain  Gain=10  OutDataTypeStr=single
  PX4 uORB Message1 : px4uORBlib/PX4 uORB Message  uORBTopic=DebugArray  SampleTime=-1  selectInstance=DebugArray
  PX4 uORB Message2 : px4uORBlib/PX4 uORB Message  uORBTopic=DebugValue  SampleTime=-1  selectInstance=DebugValue
  PX4 uORB Read1 : px4uORBlib/PX4 uORB Read  uORBTopic=DebugValue  selectInstance=DebugValue  SampleTime=-1  BlockingMode=off  BlockTimeout=1e-3
  PX4 uORB Write1 : px4uORBlib/PX4 uORB Write  uORBTopic=DebugArray  selectInstance=DebugArray  MessageQueueLen=1
  PX4 uORB Write2 : px4uORBlib/PX4 uORB Write  uORBTopic=DebugValue  selectInstance=DebugValue  MessageQueueLen=1
  Rate Transition1 : RateTransition  OutPortSampleTime=1/500
  Read debug : Scope  NumInputPorts=3
      settings: ActiveDisplayYMinimum=-0.12499999999999997  ActiveDisplayYMaximum=1.125  DataLoggingVariableName=ScopeData9
  Relational Operator : RelationalOperator  Operator=>  OutDataTypeStr=boolean  RndMeth=Simplest  InputSameDT=off
  Switch : Switch  Criteria=u2 > Threshold  SaturateOnIntegerOverflow=off  InputSameDT=off
  Debug True : Outport
  wires:
  PX4 uORB Message2/1 -> Bus Assignment2/1
  Bus Selector7/1 -> Read debug/3  "<value>"
  Relational Operator/1 -> Debug True/1, Read debug/1, Gain/1, Switch/2  "Flag"
  Constant/1 -> Relational Operator/2
  Bus Assignment2/1 -> PX4 uORB Write2/1  "bus"
  Rate Transition1/1 -> Bus Assignment2/2
  PX4 uORB Read1/2 -> Bus Selector7/1
  Gain/1 -> Rate Transition1/1
  <alt>/1 -> Relational Operator/1
  PX4 uORB Read1/1 -> Read debug/2
  PX4 uORB Message1/1 -> Bus Assignment1/1
  Constant1/1 -> Switch/3
  Constant2/1 -> Switch/1
  Switch/1 -> Bus Assignment1/2
  Bus Assignment1/1 -> PX4 uORB Write1/1  "bus"

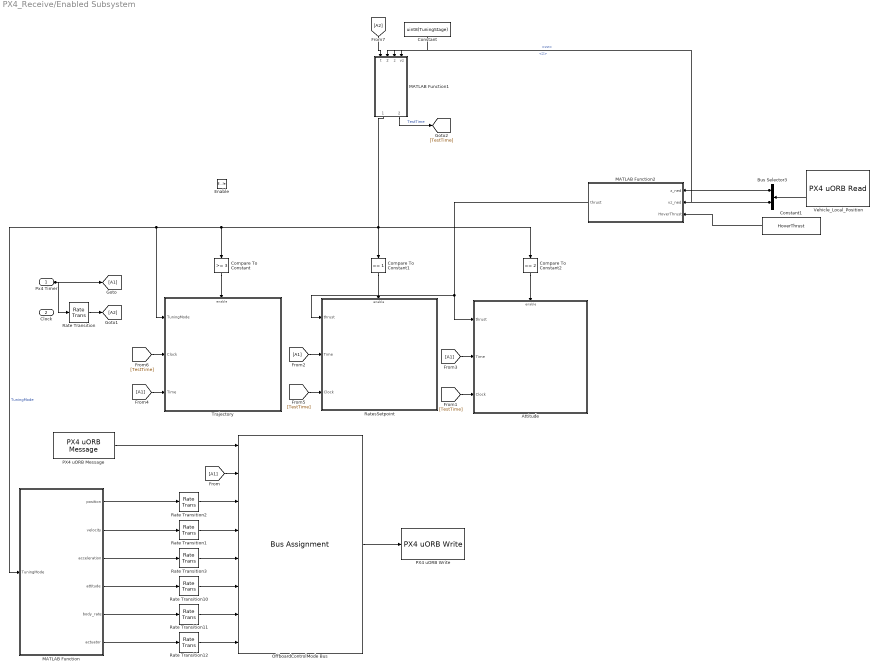
== system PX4_Receive/Enabled Subsystem ==
  Px4 Timer : Inport
  Clock : Inport  Port=2
  Enable : EnablePort
  Attitude : Subsystem
  Bus Selector3 : BusSelector  OutputSignals=z,vz
  Compare To Constant : simulink/Logic and Bit Operations/Compare To Constant  relop=>=  const=3  OutDataTypeStr=boolean
  Compare To Constant1 : simulink/Logic and Bit Operations/Compare To Constant  relop===  const=1  OutDataTypeStr=boolean
  Compare To Constant2 : simulink/Logic and Bit Operations/Compare To Constant  relop===  const=2  OutDataTypeStr=boolean
  Constant : Constant  Value=uint8(TuningStage)
  Constant1 : Constant  Value=HoverThrust
  MATLAB Function : MATLAB Function  TreatAsAtomicUnit=on
  MATLAB Function1 : MATLAB Function  TreatAsAtomicUnit=on
  MATLAB Function2 : MATLAB Function  TreatAsAtomicUnit=on
  OffboardControlMode Bus : BusAssignment  AssignedSignals=timestamp,position,velocity,acceleration,attitude,body_rate,actuator
  PX4 uORB Message : px4uORBlib/PX4 uORB Message  uORBTopic=OffboardControlMode  SampleTime=-1  selectInstance=OffboardControlMode
  PX4 uORB Write : px4uORBlib/PX4 uORB Write  uORBTopic=OffboardControlMode  selectInstance=OffboardControlMode  MessageQueueLen=1
  Rate Transition : RateTransition  OutPortSampleTime=0.01
  Rate Transition{1..3,10..12} (6 alike) : RateTransition  Deterministic=off  OutPortSampleTime=0.01
  RatesSetpoint : Subsystem
  Trajectory : Subsystem
  Vehicle_Local_Position : px4uORBlib/PX4 uORB Read  uORBTopic=VehicleLocalPosition  selectInstance=vehicle_local_position  SampleTime=-1  BlockingMode=off  BlockTimeout=1e-3
  wires:
  Rate Transition2/1 -> OffboardControlMode Bus/3
  PX4 uORB Message/1 -> OffboardControlMode Bus/1
  OffboardControlMode Bus/1 -> PX4 uORB Write/1
  MATLAB Function/3(acceleration) -> Rate Transition3/1
  MATLAB Function/1(position) -> Rate Transition2/1
  Rate Transition1/1 -> OffboardControlMode Bus/4
  Rate Transition3/1 -> OffboardControlMode Bus/5
  Rate Transition10/1 -> OffboardControlMode Bus/6
  Rate Transition11/1 -> OffboardControlMode Bus/7
  Rate Transition12/1 -> OffboardControlMode Bus/8
  MATLAB Function/6(actuator) -> Rate Transition12/1
  MATLAB Function/5(body_rate) -> Rate Transition11/1
  MATLAB Function/4(attitude) -> Rate Transition10/1
  MATLAB Function/2(velocity) -> Rate Transition1/1
  Px4 Timer/1 -> [A1], Rate Transition/1
  [A1] -> OffboardControlMode Bus/2
  MATLAB Function1/1(TuningMode) -> Compare To Constant1/1, Compare To Constant2/1, Trajectory/1(TuningMode), MATLAB Function/1(TuningMode), Compare To Constant/1  "TuningMode"
  [A1] -> RatesSetpoint/2(Time)
  [A1] -> Attitude/2(Time)
  Compare To Constant/1 -> Trajectory/Enable
  Compare To Constant1/1 -> RatesSetpoint/Enable
  Compare To Constant2/1 -> Attitude/Enable
  [TestTime] -> Trajectory/2(Clock)
  Rate Transition/1 -> [A2]
  [A2] -> MATLAB Function1/1(t)
  Constant/1 -> MATLAB Function1/2(TuningStage)
  MATLAB Function1/2(TestTime) -> [TestTime]  "TestTime"
  [TestTime] -> Attitude/3(Clock)
  [TestTime] -> RatesSetpoint/3(Clock)
  [A1] -> Trajectory/3(Time)
  Vehicle_Local_Position/2 -> Bus Selector3/1
  Bus Selector3/2 -> MATLAB Function2/2(vz_ned), MATLAB Function1/4(vz)  "<vz>"
  Bus Selector3/1 -> MATLAB Function2/1(z_ned), MATLAB Function1/3(z)  "<z>"
  Constant1/1 -> MATLAB Function2/3(HoverThrust)
  MATLAB Function2/1(thrust) -> Attitude/1(thrust), RatesSetpoint/1(thrust)

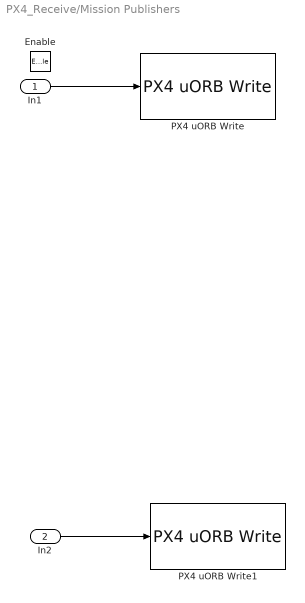
== system PX4_Receive/Mission Publishers ==
  In1 : Inport
  In2 : Inport  Port=2
  Enable : EnablePort
  PX4 uORB Write : px4uORBlib/PX4 uORB Write  uORBTopic=OffboardControlMode  selectInstance=OffboardControlMode  MessageQueueLen=1
  PX4 uORB Write1 : px4uORBlib/PX4 uORB Write  uORBTopic=TrajectorySetpoint  selectInstance=TrajectorySetpoint  MessageQueueLen=1
  wires:
  In2/1 -> PX4 uORB Write1/1
  In1/1 -> PX4 uORB Write/1
